simulink model "soc_02_kalman_filter"  (R2025a)
settings: Solver=FixedStepDiscrete  StartTime=0.0  StopTime=240  FixedStep=1  RelTol=1e-3
undefined symbols (not defined in the file): DiscIntNeverNeededParam
Description:
  | Lesson 2: Use terminal voltage to correct the SOC prediction. The battery starts at 80%; both estimators start at 50%. Open Predict and correct to read the two steps. The noise seed is fixed.
settings Model: Creator=mosri  LastModifiedBy=mosri

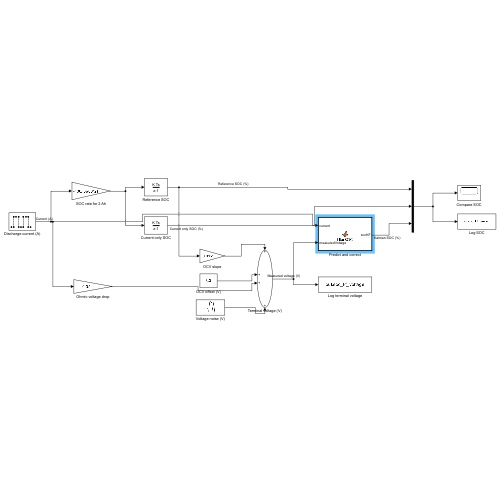
[thumbnail: Simulink's stored preview of the top-level diagram]
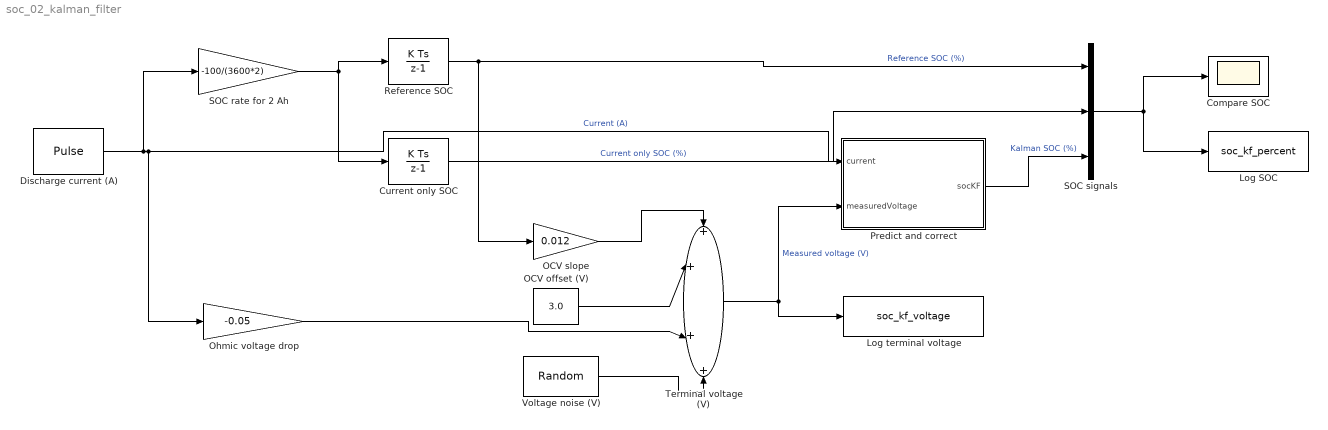
== system soc_02_kalman_filter ==
  Compare SOC : Scope
      settings: Title=Reference, current only, and Kalman filter  ActiveDisplayYMinimum=45  ActiveDisplayYMaximum=85  YLabel=SOC (%)
  Current only SOC : DiscreteIntegrator  InitialCondition=50  ICPrevOutput=DiscIntNeverNeededParam  ICPrevScaledInput=DiscIntNeverNeededParam
  Discharge current (A) : DiscretePulseGenerator  Period=120  PulseWidth=60
  Log SOC : ToWorkspace  VariableName=soc_kf_percent  SampleTime=-1
  Log terminal voltage : ToWorkspace  VariableName=soc_kf_voltage  SampleTime=-1
  OCV offset (V) : Constant  Value=3.0
  OCV slope : Gain  Gain=0.012
  Ohmic voltage drop : Gain  Gain=-0.05
  Predict and correct : MATLAB Function  TreatAsAtomicUnit=on
  Reference SOC : DiscreteIntegrator  InitialCondition=80  ICPrevOutput=DiscIntNeverNeededParam  ICPrevScaledInput=DiscIntNeverNeededParam
  SOC rate for 2 Ah : Gain  Gain=-100/(3600*2)
  SOC signals : Mux  Inputs=3
  Terminal voltage (V) : Sum  Inputs=++++
  Voltage noise (V) : RandomNumber  Variance=0.02^2  Seed=42  SampleTime=1
  wires:
  Discharge current (A)/1 -> Ohmic voltage drop/1, Predict and correct/1(current), SOC rate for 2 Ah/1  "Current (A)"
  SOC rate for 2 Ah/1 -> Reference SOC/1, Current only SOC/1
  Reference SOC/1 -> SOC signals/1, OCV slope/1  "Reference SOC (%)"
  Current only SOC/1 -> SOC signals/2  "Current only SOC (%)"
  OCV slope/1 -> Terminal voltage (V)/1
  OCV offset (V)/1 -> Terminal voltage (V)/2
  Ohmic voltage drop/1 -> Terminal voltage (V)/3
  Voltage noise (V)/1 -> Terminal voltage (V)/4
  Terminal voltage (V)/1 -> Predict and correct/2(measuredVoltage), Log terminal voltage/1  "Measured voltage (V)"
  Predict and correct/1(socKF) -> SOC signals/3  "Kalman SOC (%)"
  SOC signals/1 -> Compare SOC/1, Log SOC/1

== matlab function soc_02_kalman_filter/Predict and correct ==
  data: current input; socKF output; measuredVoltage input
function socKF = filterSOC(current, measuredVoltage)
% SOC is in percent. Current is positive during discharge.
persistent soc P previousCurrent
if isempty(soc)
    soc = 50;
    P = 5^2;                 % Initial SOC error variance (percentage points squared)
    previousCurrent = current;
    socKF = soc;
    return
end

% 1. Predict SOC from the previous 1-second interval.
socPred = soc - 100*previousCurrent/(3600*2);
pPred = P + 1e-3;             % Process noise variance per sample

% 2. Correct with the measured terminal voltage.
H = 0.012;                    % OCV slope (volts per percentage point)
R = 0.02^2;                   % Voltage measurement variance (V^2)
predictedVoltage = 3.0 + H*socPred - 0.05*current;
innovation = measuredVoltage - predictedVoltage;
K = pPred*H/(H^2*pPred + R);

soc = socPred + K*innovation;
P = (1 - K*H)*pPred;
previousCurrent = current;
socKF = soc;
end
